simulink model "case_03_fast_no_cbf"  (R2025b)
settings: Solver=VariableStepAuto  StartTime=0.0  StopTime=60  RelTol=1e-3
settings Model: Creator=sanborkl  LastModifiedBy=sanborkl

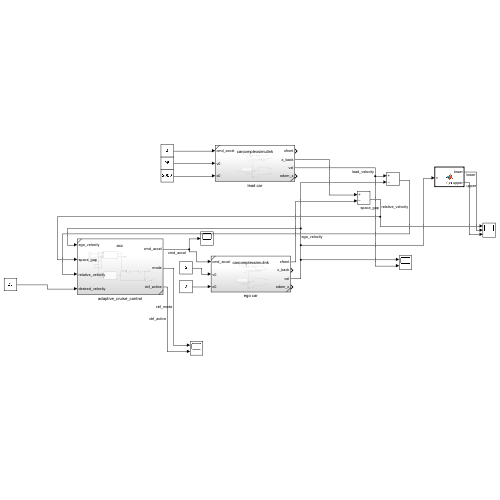
[thumbnail: Simulink's stored preview of the top-level diagram]
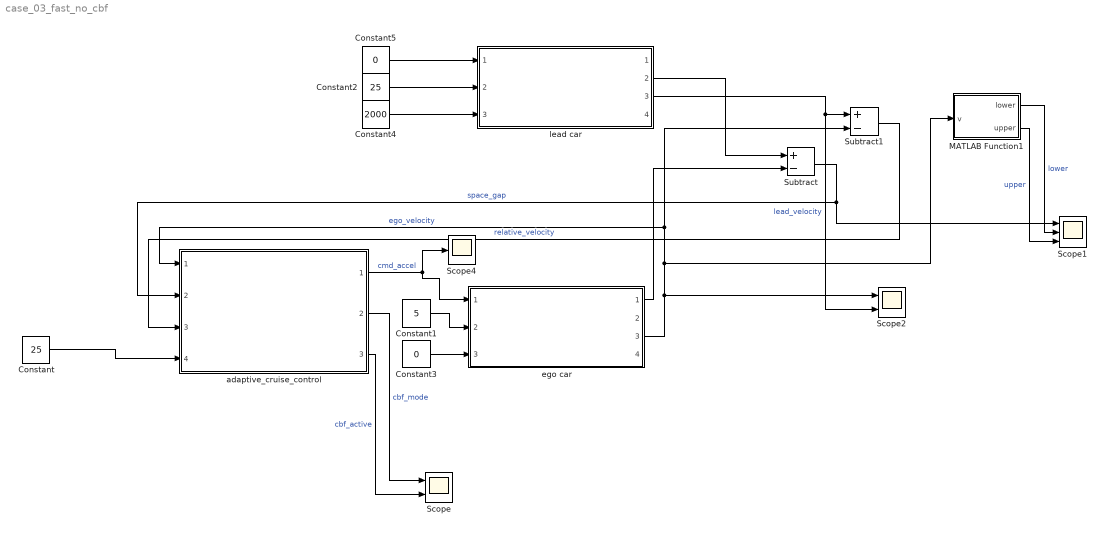
== system case_03_fast_no_cbf ==
  Constant : Constant  Value=25
  Constant1 : Constant  Value=5
  Constant2 : Constant  Value=25
  Constant3 : Constant  Value=0
  Constant4 : Constant  Value=2000
  Constant5 : Constant  Value=0
  MATLAB Function1 : MATLAB Function  TreatAsAtomicUnit=on
  Scope : Scope  NumInputPorts=2
      settings: ActiveDisplayYMinimum=0.9  ActiveDisplayYMaximum=1.1
  Scope1 : Scope  NumInputPorts=3
      settings: ActiveDisplayYMinimum=-250.91478956902256  ActiveDisplayYMaximum=2408.2331061212035  YLabel=m
  Scope2 : Scope  NumInputPorts=2
      settings: ActiveDisplayYMinimum=2.4969765535388997  ActiveDisplayYMaximum=27.527211018149909  YLabel=m/s  DataLoggingVariableName=ScopeData2
  Scope4 : Scope
      settings: ActiveDisplayYMinimum=-1  ActiveDisplayYMaximum=1  YLabel=m/s^2  DataLoggingVariableName=ScopeData6
  Subtract : Sum  Inputs=+-
  Subtract1 : Sum  Inputs=+-
  adaptive_cruise_control : Subsystem  ReferencedSubsystem=acc
  ego car : Subsystem  ReferencedSubsystem=carcomplexsimulink
  lead car : Subsystem  ReferencedSubsystem=carcomplexsimulink
  wires:
  Constant4/1 -> lead car/3
  Subtract/1 -> Scope1/1, adaptive_cruise_control/2  "space_gap"
  Constant2/1 -> lead car/2
  Constant1/1 -> ego car/2
  lead car/3 -> Scope2/2, Subtract1/1  "lead_velocity"
  MATLAB Function1/1(lower) -> Scope1/2  "lower"
  adaptive_cruise_control/2 -> Scope/1  "cbf_mode"
  Constant3/1 -> ego car/3
  Constant/1 -> adaptive_cruise_control/4
  ego car/1 -> Subtract/2
  Subtract1/1 -> adaptive_cruise_control/3  "relative_velocity"
  MATLAB Function1/2(upper) -> Scope1/3  "upper"
  adaptive_cruise_control/3 -> Scope/2  "cbf_active"
  adaptive_cruise_control/1 -> ego car/1, Scope4/1  "cmd_accel"
  ego car/3 -> Subtract1/2, adaptive_cruise_control/1, MATLAB Function1/1(v), Scope2/1  "ego_velocity"
  Constant5/1 -> lead car/1
  lead car/2 -> Subtract/1

== matlab function case_03_fast_no_cbf/MATLAB Function1 ==
  data: v input; lower output; upper output
function [lower, upper] = fcn(v)

lower = 2 * v + 5;
upper = 2 * v + 15;
